simulink model "mano_buena_pinza_paper"  (R2025a)
settings: Solver=ode23  StartTime=0.0  StopTime=10.5  FixedStep=20e-3  MaxStep=1e-3  RelTol=1e-2  AbsTol=1e-4
model workspace: external: MATLAB File mano_vf_DataFile1.m (data not in the file)
undefined symbols (not defined in the file): smiData, X, Y, Z
libraries: sm_lib x268, nesl_utility x26
(part 3 of 7)

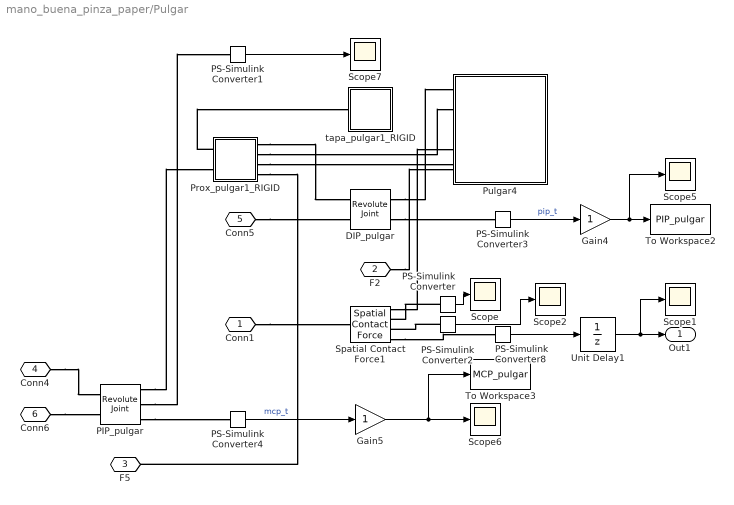
== system mano_buena_pinza_paper/Pulgar ==
  DIP_pulgar : sm_lib/Joints/Revolute Joint  JointMode=Normal  CompositeWrenchDir=FollowerOnBase  CompositeWrenchFrame=BaseFrame  SenseConstraintForce=off  SenseConstraintTorque=off  SenseTotalForce=off  SenseTotalTorque=off  PositionTargetSpecify=on  PositionTargetPriority=Low  PositionTargetValue=smiData.RevoluteJoint(41).Rz.Pos  PositionTargetValueUnits=deg  VelocityTargetSpecify=off  VelocityTargetPriority=High  VelocityTargetValue=0  VelocityTargetValueUnits=deg/s  EquilibriumPosition=0  EquilibriumPositionUnits=deg  SpringStiffness=0  SpringStiffnessUnits=N*m/deg  DampingCoefficient=0  DampingCoefficientUnits=N*m/(deg/s)  LowerLimitSpecify=off  LowerLimitBound=-90  LowerLimitBoundUnits=deg  LowerLimitStiffness=1e4  LowerLimitStiffnessUnits=N*m/deg  LowerLimitDamping=10  LowerLimitDampingUnits=N*m/(deg/s)  LowerLimitTransitionRegionWidth=0.1  LowerLimitTransitionRegionWidthUnits=deg  UpperLimitSpecify=off  UpperLimitBound=90  UpperLimitBoundUnits=deg  UpperLimitStiffness=1e4  UpperLimitStiffnessUnits=N*m/deg  UpperLimitDamping=10  UpperLimitDampingUnits=N*m/(deg/s)  UpperLimitTransitionRegionWidth=0.1  UpperLimitTransitionRegionWidthUnits=deg  TorqueActuationMode=ComputedTorque  MotionActuationMode=InputMotion  SensePosition=off  SenseVelocity=off  SenseAcceleration=off  SenseTorqueForce=on  SenseLowerLimitTorqueForce=off  SenseUpperLimitTorqueForce=off
  Gain4 : Gain
  Gain5 : Gain
  PIP_pulgar : sm_lib/Joints/Revolute Joint  JointMode=Normal  CompositeWrenchDir=FollowerOnBase  CompositeWrenchFrame=BaseFrame  SenseConstraintForce=off  SenseConstraintTorque=off  SenseTotalForce=off  SenseTotalTorque=off  PositionTargetSpecify=on  PositionTargetPriority=Low  PositionTargetValue=smiData.RevoluteJoint(36).Rz.Pos  PositionTargetValueUnits=deg  VelocityTargetSpecify=off  VelocityTargetPriority=High  VelocityTargetValue=0  VelocityTargetValueUnits=deg/s  EquilibriumPosition=0  EquilibriumPositionUnits=deg  SpringStiffness=0  SpringStiffnessUnits=N*m/deg  DampingCoefficient=0  DampingCoefficientUnits=N*m/(deg/s)  LowerLimitSpecify=off  LowerLimitBound=-90  LowerLimitBoundUnits=deg  LowerLimitStiffness=1e4  LowerLimitStiffnessUnits=N*m/deg  LowerLimitDamping=10  LowerLimitDampingUnits=N*m/(deg/s)  LowerLimitTransitionRegionWidth=0.1  LowerLimitTransitionRegionWidthUnits=deg  UpperLimitSpecify=off  UpperLimitBound=90  UpperLimitBoundUnits=deg  UpperLimitStiffness=1e4  UpperLimitStiffnessUnits=N*m/deg  UpperLimitDamping=10  UpperLimitDampingUnits=N*m/(deg/s)  UpperLimitTransitionRegionWidth=0.1  UpperLimitTransitionRegionWidthUnits=deg  TorqueActuationMode=ComputedTorque  MotionActuationMode=InputMotion  SensePosition=on  SenseVelocity=off  SenseAcceleration=off  SenseTorqueForce=on  SenseLowerLimitTorqueForce=off  SenseUpperLimitTorqueForce=off
  PS-Simulink Converter : nesl_utility/PS-Simulink Converter  PhysicalDomain=network_engine_domain  SubClassName=ps_output  LeftPortType=input  RightPortType=output  PseudoPeriodic=off  Frequencies=[]  VectorFormat=inherit  Unit=inherit  AffineConversion=off
  PS-Simulink Converter1 : nesl_utility/PS-Simulink Converter  PhysicalDomain=network_engine_domain  SubClassName=ps_output  LeftPortType=input  RightPortType=output  PseudoPeriodic=off  Frequencies=[]  VectorFormat=inherit  Unit=deg  AffineConversion=off
  PS-Simulink Converter2 : nesl_utility/PS-Simulink Converter  PhysicalDomain=network_engine_domain  SubClassName=ps_output  LeftPortType=input  RightPortType=output  PseudoPeriodic=off  Frequencies=[]  VectorFormat=inherit  Unit=mm  AffineConversion=off
  PS-Simulink Converter3 : nesl_utility/PS-Simulink Converter  PhysicalDomain=network_engine_domain  SubClassName=ps_output  LeftPortType=input  RightPortType=output  PseudoPeriodic=off  Frequencies=[]  VectorFormat=inherit  Unit=N*mm  AffineConversion=off
  PS-Simulink Converter4 : nesl_utility/PS-Simulink Converter  PhysicalDomain=network_engine_domain  SubClassName=ps_output  LeftPortType=input  RightPortType=output  PseudoPeriodic=off  Frequencies=[]  VectorFormat=inherit  Unit=N*mm  AffineConversion=off
  PS-Simulink Converter8 : nesl_utility/PS-Simulink Converter  PhysicalDomain=network_engine_domain  SubClassName=ps_output  LeftPortType=input  RightPortType=output  PseudoPeriodic=off  Frequencies=[]  VectorFormat=inherit  Unit=N  AffineConversion=off
  Prox_pulgar1_RIGID : Subsystem
  Pulgar4 : Subsystem
  Scope{,1..2,5..7} (6 alike) : Scope
      Scope settings: DataLoggingVariableName=ScopeData15
      Scope1 settings: ActiveDisplayYMinimum=-0.19095791938029771  ActiveDisplayYMaximum=2.3213655450923372
      Scope2 settings: DataLoggingVariableName=ScopeData16
      Scope5 settings: ActiveDisplayYMinimum=-74.001415056347014  ActiveDisplayYMaximum=341.55104024365312  DataLoggingVariableName=ScopeData5
      Scope6 settings: ActiveDisplayYMinimum=-154.71464722510333  ActiveDisplayYMaximum=184.74085697959597  DataLoggingVariableName=ScopeData6
      Scope7 settings: ActiveDisplayYMinimum=-1  ActiveDisplayYMaximum=1  DataLoggingVariableName=ScopeData7
  Spatial Contact Force1 : sm_lib/Forces and Torques/Spatial Contact Force  SenseSeparationDistance=off  NormalForceType=SmoothSpringDamper  NormalStiffness=2e4  NormalStiffnessUnits=N/m  NormalDamping=30  NormalDampingUnits=N/(m/s)  NormalTransitionRegionWidth=1e-3  NormalTransitionRegionWidthUnits=m  FrictionType=SmoothStickSlip  CoefficientOfStaticFriction=0.5  CoefficientOfDynamicFriction=0.3  FrictionalCriticalVelocity=1e-2  FrictionalCriticalVelocityUnits=m/s  SenseContactSignal=on  SensePenetrationDepth=on  SenseNormalVelocity=off  SenseTangentialVelocity=off  SensingForceTorqueDirection=BaseOnFollower  SensingForceTorqueResolutionFrame=ContactFrame  SenseNormalForce=off  SenseNormalForceMagnitude=on  SenseNormalTorque=off  SenseFrictionalForce=off  SenseFrictionalForceMagnitude=off  SenseFrictionalTorque=off  SenseTotalForce=off  SenseTotalTorque=off  SenseContactBaseRotation=off  SenseContactBaseTranslation=off  SenseContactFollowerRotation=off  SenseContactFollowerTranslation=off  ZeroCrossDetectContactStartAndEnd=off
  To Workspace2 : ToWorkspace  VariableName=PIP_pulgar  SaveFormat=Timeseries  SampleTime=-1
  To Workspace3 : ToWorkspace  VariableName=MCP_pulgar  SaveFormat=Timeseries  SampleTime=-1
  Unit Delay1 : UnitDelay  SampleTime=20e-3  HasFrameUpgradeWarning=on
  tapa_pulgar1_RIGID : Subsystem
  Conn1 : PMIOPort  Side=Left
  F2 : PMIOPort  Port=2  Side=Left
  F5 : PMIOPort  Port=3  Side=Right
  Conn4 : PMIOPort  Port=4  Side=Left
  Conn5 : PMIOPort  Port=5  Side=Left
  Conn6 : PMIOPort  Port=6  Side=Left
  Out1 : Outport
  wires:
  PS-Simulink Converter1/1 -> Scope7/1
  PS-Simulink Converter4/1 -> Gain5/1  "mcp_t"
  Gain5/1 -> To Workspace3/1, Scope6/1
  PS-Simulink Converter3/1 -> Gain4/1  "pip_t"
  PS-Simulink Converter8/1 -> Unit Delay1/1
  Gain4/1 -> To Workspace2/1, Scope5/1
  Unit Delay1/1 -> Scope1/1, Out1/1
  PS-Simulink Converter/1 -> Scope/1
  PS-Simulink Converter2/1 -> Scope2/1
  connections:
  Conn6/RConn1 -- PIP_pulgar/LConn2
  Conn4/RConn1 -- PIP_pulgar/LConn1
  DIP_pulgar/RConn1 -- Pulgar4/LConn1
  Prox_pulgar1_RIGID/LConn1 -- tapa_pulgar1_RIGID/LConn1
  PIP_pulgar/RConn1 -- Prox_pulgar1_RIGID/LConn2
  PIP_pulgar/RConn2 -- PS-Simulink Converter1/LConn1
  Prox_pulgar1_RIGID/RConn1 -- DIP_pulgar/LConn1
  PIP_pulgar/RConn3 -- PS-Simulink Converter4/LConn1
  Prox_pulgar1_RIGID/RConn4 -- F5/RConn1
  Prox_pulgar1_RIGID/RConn2 -- Pulgar4/LConn2
  Prox_pulgar1_RIGID/RConn3 -- Pulgar4/LConn3
  Conn5/RConn1 -- DIP_pulgar/LConn2
  Conn1/RConn1 -- Spatial Contact Force1/LConn1
  DIP_pulgar/RConn2 -- PS-Simulink Converter3/LConn1
  F2/RConn1 -- Pulgar4/LConn5
  Spatial Contact Force1/RConn1 -- Pulgar4/LConn4
  Spatial Contact Force1/RConn4 -- PS-Simulink Converter8/LConn1
  PS-Simulink Converter/LConn1 -- Spatial Contact Force1/RConn2
  PS-Simulink Converter2/LConn1 -- Spatial Contact Force1/RConn3

== system mano_buena_pinza_paper/Subsystem ==
  Angulo_ref : Inport
  Demux1 : Demux  Outputs=2
  Discrete State-Space : DiscreteStateSpace  A=[1 0.0196;0 0.9604]  B=[1e-4*0.0051;1e-4*0.5045]  C=eye(2)  D=[0 ;0]  SampleTime=20e-3
  Gain : Gain  Gain=pi/180
  Gain1 : Gain  Gain=1000
  Gain4 : Gain  Gain=180/pi
  Gain5 : Gain  Gain=[2192.4 757.4]  Multiplication=Matrix(K*u) (u vector)
  Saturation : Saturate  UpperLimit=4095  LowerLimit=-4095
  Scope1 : Scope
      settings: ActiveDisplayYMinimum=-514.3876517918344  ActiveDisplayYMaximum=3883.614035604794  DataLoggingVariableName=ScopeData8
  Scope6 : Scope
      settings: ActiveDisplayYMinimum=-70.37229560740974  ActiveDisplayYMaximum=586.35935668183049  DataLoggingVariableName=ScopeData11
  Sum : Sum  Inputs=|+-
  Angulo_real : Outport
  wires:
  Gain5/1 -> Saturation/1
  Discrete State-Space/1 -> Demux1/1, Sum/2  "LQR"
  Sum/1 -> Gain5/1
  Saturation/1 -> Scope1/1, Discrete State-Space/1
  Demux1/1 -> Gain4/1
  Angulo_ref/1 -> Gain/1
  Demux1/2 -> Gain1/1
  Gain4/1 -> Angulo_real/1
  Gain/1 -> Sum/1
  Gain1/1 -> Scope6/1

== system mano_buena_pinza_paper/Subsystem1 ==
  Angulo_ref : Inport
  Demux1 : Demux  Outputs=2
  Discrete State-Space : DiscreteStateSpace  A=[1 0.0196;0 0.9604]  B=[1e-4*0.0051;1e-4*0.5045]  C=eye(2)  D=[0 ;0]  SampleTime=20e-3
  Gain : Gain  Gain=pi/180
  Gain1 : Gain  Gain=1000
  Gain4 : Gain  Gain=180/pi
  Gain5 : Gain  Gain=[2192.4 757.4]  Multiplication=Matrix(K*u) (u vector)
  Saturation : Saturate  UpperLimit=4095  LowerLimit=-4095
  Scope1 : Scope
      settings: ActiveDisplayYMinimum=-514.3876517918344  ActiveDisplayYMaximum=3883.614035604794  DataLoggingVariableName=ScopeData8
  Scope6 : Scope
      settings: ActiveDisplayYMinimum=-178.26281177195131  ActiveDisplayYMaximum=1149.4351414549326  DataLoggingVariableName=ScopeData11
  Sum : Sum  Inputs=|+-
  Angulo_real : Outport
  wires:
  Gain5/1 -> Saturation/1
  Discrete State-Space/1 -> Demux1/1, Sum/2  "LQR"
  Sum/1 -> Gain5/1
  Saturation/1 -> Scope1/1, Discrete State-Space/1
  Demux1/1 -> Gain4/1
  Angulo_ref/1 -> Gain/1
  Demux1/2 -> Gain1/1
  Gain4/1 -> Angulo_real/1
  Gain/1 -> Sum/1
  Gain1/1 -> Scope6/1

== system mano_buena_pinza_paper/Subsystem2 ==
  Angulo_ref : Inport
  Demux1 : Demux  Outputs=2
  Discrete State-Space : DiscreteStateSpace  A=[1 0.0196;0 0.9604]  B=[1e-4*0.0051;1e-4*0.5045]  C=eye(2)  D=[0 ;0]  SampleTime=20e-3
  Gain : Gain  Gain=pi/180
  Gain4 : Gain  Gain=180/pi
  Gain5 : Gain  Gain=[2192.4 757.4]  Multiplication=Matrix(K*u) (u vector)
  Saturation : Saturate  UpperLimit=4095  LowerLimit=-4095
  Scope1 : Scope
      settings: ActiveDisplayYMinimum=-514.3876517918344  ActiveDisplayYMaximum=3883.614035604794  DataLoggingVariableName=ScopeData8
  Scope6 : Scope
      settings: ActiveDisplayYMinimum=-0.21091417850221092  ActiveDisplayYMaximum=1.7573278410890731  DataLoggingVariableName=ScopeData11
  Sum : Sum  Inputs=|+-
  Angulo_real : Outport
  wires:
  Gain5/1 -> Saturation/1
  Discrete State-Space/1 -> Demux1/1, Sum/2  "LQR"
  Sum/1 -> Gain5/1
  Saturation/1 -> Scope1/1, Discrete State-Space/1
  Demux1/1 -> Gain4/1
  Angulo_ref/1 -> Gain/1
  Demux1/2 -> Scope6/1
  Gain4/1 -> Angulo_real/1
  Gain/1 -> Sum/1

== system mano_buena_pinza_paper/Subsystem3 ==
  Angulo_ref : Inport
  Demux1 : Demux  Outputs=2
  Discrete State-Space : DiscreteStateSpace  A=[1 0.0196;0 0.9604]  B=[1e-4*0.0051;1e-4*0.5045]  C=eye(2)  D=[0 ;0]  SampleTime=20e-3
  Gain : Gain  Gain=pi/180
  Gain4 : Gain  Gain=180/pi
  Gain5 : Gain  Gain=[2192.4 757.4]  Multiplication=Matrix(K*u) (u vector)
  Saturation : Saturate  UpperLimit=4095  LowerLimit=-4095
  Scope1 : Scope
      settings: ActiveDisplayYMinimum=-514.3876517918344  ActiveDisplayYMaximum=3883.614035604794  DataLoggingVariableName=ScopeData8
  Scope6 : Scope
      settings: ActiveDisplayYMinimum=-0.21091417850221092  ActiveDisplayYMaximum=1.7573278410890731  DataLoggingVariableName=ScopeData11
  Sum : Sum  Inputs=|+-
  Angulo_real : Outport
  wires:
  Gain5/1 -> Saturation/1
  Discrete State-Space/1 -> Demux1/1, Sum/2  "LQR"
  Sum/1 -> Gain5/1
  Saturation/1 -> Scope1/1, Discrete State-Space/1
  Demux1/1 -> Gain4/1
  Angulo_ref/1 -> Gain/1
  Demux1/2 -> Scope6/1
  Gain4/1 -> Angulo_real/1
  Gain/1 -> Sum/1

== system mano_buena_pinza_paper/Subsystem4 ==
  Angulo_ref : Inport
  Demux1 : Demux  Outputs=2
  Discrete State-Space : DiscreteStateSpace  A=[1 0.0196;0 0.9604]  B=[1e-4*0.0051;1e-4*0.5045]  C=eye(2)  D=[0 ;0]  SampleTime=20e-3
  Gain : Gain  Gain=pi/180
  Gain4 : Gain  Gain=180/pi
  Gain5 : Gain  Gain=[2192.4 757.4]  Multiplication=Matrix(K*u) (u vector)
  Saturation : Saturate  UpperLimit=4095  LowerLimit=-4095
  Scope1 : Scope
      settings: ActiveDisplayYMinimum=-514.3876517918344  ActiveDisplayYMaximum=3883.614035604794  DataLoggingVariableName=ScopeData8
  Scope6 : Scope
      settings: ActiveDisplayYMinimum=-0.21091417850221092  ActiveDisplayYMaximum=1.7573278410890731  DataLoggingVariableName=ScopeData11
  Sum : Sum  Inputs=|+-
  Angulo_real : Outport
  wires:
  Gain5/1 -> Saturation/1
  Discrete State-Space/1 -> Demux1/1, Sum/2  "LQR"
  Sum/1 -> Gain5/1
  Saturation/1 -> Scope1/1, Discrete State-Space/1
  Demux1/1 -> Gain4/1
  Angulo_ref/1 -> Gain/1
  Demux1/2 -> Scope6/1
  Gain4/1 -> Angulo_real/1
  Gain/1 -> Sum/1

== system mano_buena_pinza_paper/Subsystem5 ==
  Angulo_ref : Inport
  Demux1 : Demux  Outputs=2
  Discrete State-Space : DiscreteStateSpace  A=[1 0.0196;0 0.9604]  B=[1e-4*0.0051;1e-4*0.5045]  C=eye(2)  D=[0 ;0]  SampleTime=20e-3
  Gain : Gain  Gain=pi/180
  Gain4 : Gain  Gain=180/pi
  Gain5 : Gain  Gain=[2192.4 757.4]  Multiplication=Matrix(K*u) (u vector)
  Saturation : Saturate  UpperLimit=4095  LowerLimit=-4095
  Scope1 : Scope
      settings: ActiveDisplayYMinimum=-514.3876517918344  ActiveDisplayYMaximum=3883.614035604794  DataLoggingVariableName=ScopeData8
  Scope6 : Scope
      settings: ActiveDisplayYMinimum=-0.21091417850221092  ActiveDisplayYMaximum=1.7573278410890731  DataLoggingVariableName=ScopeData11
  Sum : Sum  Inputs=|+-
  Angulo_real : Outport
  wires:
  Gain5/1 -> Saturation/1
  Discrete State-Space/1 -> Demux1/1, Sum/2  "LQR"
  Sum/1 -> Gain5/1
  Saturation/1 -> Scope1/1, Discrete State-Space/1
  Demux1/1 -> Gain4/1
  Angulo_ref/1 -> Gain/1
  Demux1/2 -> Scope6/1
  Gain4/1 -> Angulo_real/1
  Gain/1 -> Sum/1

== system mano_buena_pinza_paper/Subsystem6 ==
  Angulo_ref : Inport
  Demux1 : Demux  Outputs=2
  Discrete State-Space : DiscreteStateSpace  A=[1 0.0196;0 0.9604]  B=[1e-4*0.0051;1e-4*0.5045]  C=eye(2)  D=[0 ;0]  SampleTime=20e-3
  Gain : Gain  Gain=pi/180
  Gain4 : Gain  Gain=180/pi
  Gain5 : Gain  Gain=[2192.4 757.4]  Multiplication=Matrix(K*u) (u vector)
  Saturation : Saturate  UpperLimit=4095  LowerLimit=-4095
  Scope1 : Scope
      settings: ActiveDisplayYMinimum=-514.3876517918344  ActiveDisplayYMaximum=3883.614035604794  DataLoggingVariableName=ScopeData8
  Scope6 : Scope
      settings: ActiveDisplayYMinimum=-0.21091417850221092  ActiveDisplayYMaximum=1.7573278410890731  DataLoggingVariableName=ScopeData11
  Sum : Sum  Inputs=|+-
  Angulo_real : Outport
  wires:
  Gain5/1 -> Saturation/1
  Discrete State-Space/1 -> Demux1/1, Sum/2  "LQR"
  Sum/1 -> Gain5/1
  Saturation/1 -> Scope1/1, Discrete State-Space/1
  Demux1/1 -> Gain4/1
  Angulo_ref/1 -> Gain/1
  Demux1/2 -> Scope6/1
  Gain4/1 -> Angulo_real/1
  Gain/1 -> Sum/1

== system mano_buena_pinza_paper/Subsystem7 ==
  Angulo_ref : Inport
  Demux1 : Demux  Outputs=2
  Discrete State-Space : DiscreteStateSpace  A=[1 0.0196;0 0.9604]  B=[1e-4*0.0051;1e-4*0.5045]  C=eye(2)  D=[0 ;0]  SampleTime=20e-3
  Gain : Gain  Gain=pi/180
  Gain4 : Gain  Gain=180/pi
  Gain5 : Gain  Gain=[2192.4 757.4]  Multiplication=Matrix(K*u) (u vector)
  Saturation : Saturate  UpperLimit=4095  LowerLimit=-4095
  Scope1 : Scope
      settings: ActiveDisplayYMinimum=-514.3876517918344  ActiveDisplayYMaximum=3883.614035604794  DataLoggingVariableName=ScopeData8
  Scope6 : Scope
      settings: ActiveDisplayYMinimum=-0.21091417850221092  ActiveDisplayYMaximum=1.7573278410890731  DataLoggingVariableName=ScopeData11
  Sum : Sum  Inputs=|+-
  Angulo_real : Outport
  wires:
  Gain5/1 -> Saturation/1
  Discrete State-Space/1 -> Demux1/1, Sum/2  "LQR"
  Sum/1 -> Gain5/1
  Saturation/1 -> Scope1/1, Discrete State-Space/1
  Demux1/1 -> Gain4/1
  Angulo_ref/1 -> Gain/1
  Demux1/2 -> Scope6/1
  Gain4/1 -> Angulo_real/1
  Gain/1 -> Sum/1

== system mano_buena_pinza_paper/Subsystem8 ==
  Angulo_ref : Inport
  Demux1 : Demux  Outputs=2
  Discrete State-Space : DiscreteStateSpace  A=[1 0.0196;0 0.9604]  B=[1e-4*0.0051;1e-4*0.5045]  C=eye(2)  D=[0 ;0]  SampleTime=20e-3
  Gain : Gain  Gain=pi/180
  Gain4 : Gain  Gain=180/pi
  Gain5 : Gain  Gain=[2192.4 757.4]  Multiplication=Matrix(K*u) (u vector)
  Saturation : Saturate  UpperLimit=4095  LowerLimit=-4095
  Scope1 : Scope
      settings: ActiveDisplayYMinimum=-514.3876517918344  ActiveDisplayYMaximum=3883.614035604794  DataLoggingVariableName=ScopeData8
  Scope6 : Scope
      settings: ActiveDisplayYMinimum=-0.21091417850221092  ActiveDisplayYMaximum=1.7573278410890731  DataLoggingVariableName=ScopeData11
  Sum : Sum  Inputs=|+-
  Angulo_real : Outport
  wires:
  Gain5/1 -> Saturation/1
  Discrete State-Space/1 -> Demux1/1, Sum/2  "LQR"
  Sum/1 -> Gain5/1
  Saturation/1 -> Scope1/1, Discrete State-Space/1
  Demux1/1 -> Gain4/1
  Angulo_ref/1 -> Gain/1
  Demux1/2 -> Scope6/1
  Gain4/1 -> Angulo_real/1
  Gain/1 -> Sum/1

== system mano_buena_pinza_paper/Subsystem9 ==
  Angulo_ref : Inport
  Demux1 : Demux  Outputs=2
  Discrete State-Space : DiscreteStateSpace  A=[1 0.0196;0 0.9604]  B=[1e-4*0.0051;1e-4*0.5045]  C=eye(2)  D=[0 ;0]  SampleTime=20e-3
  Gain : Gain  Gain=pi/180
  Gain4 : Gain  Gain=180/pi
  Gain5 : Gain  Gain=[2192.4 757.4]  Multiplication=Matrix(K*u) (u vector)
  Saturation : Saturate  UpperLimit=4095  LowerLimit=-4095
  Scope1 : Scope
      settings: ActiveDisplayYMinimum=-514.3876517918344  ActiveDisplayYMaximum=3883.614035604794  DataLoggingVariableName=ScopeData8
  Scope6 : Scope
      settings: ActiveDisplayYMinimum=-0.21091417850221092  ActiveDisplayYMaximum=1.7573278410890731  DataLoggingVariableName=ScopeData11
  Sum : Sum  Inputs=|+-
  Angulo_real : Outport
  wires:
  Gain5/1 -> Saturation/1
  Discrete State-Space/1 -> Demux1/1, Sum/2  "LQR"
  Sum/1 -> Gain5/1
  Saturation/1 -> Scope1/1, Discrete State-Space/1
  Demux1/1 -> Gain4/1
  Angulo_ref/1 -> Gain/1
  Demux1/2 -> Scope6/1
  Gain4/1 -> Angulo_real/1
  Gain/1 -> Sum/1

== system mano_buena_pinza_paper/Tapa_meta_indice2_RIGID ==
  ReferenceFrame : sm_lib/Frames and Transforms/Reference Frame
  Solid : sm_lib/Body Elements/File Solid  ExtGeomFileName=Tapa_meta_indice_ipt_ad682b4a.STEP  UnitType=FromFile  ExtGeomFileUnits=m  StepReaderType=HEX  ExportConvexHullGeometry=off  InertiaType=Custom  BasedOnType=DensityFromFile  Density=1000  DensityUnits=kg/m^3  Mass=smiData.Solid(12).mass  MassUnits=kg  CenterOfMass=smiData.Solid(12).CoM  CenterOfMassUnits=mm  MomentsOfInertia=smiData.Solid(12).MoI  MomentsOfInertiaUnits=kg*mm^2  ProductsOfInertia=smiData.Solid(12).PoI  ProductsOfInertiaUnits=kg*mm^2  GraphicType=FromGeometry  MarkerShape=Sphere  MarkerSize=10  GraphicVisPropType=SimpleVisualProperties  GraphicDiffuseColor=smiData.Solid(12).color  GraphicOpacity=smiData.Solid(12).opacity  GraphicSpecularColor=[0.5 0.5 0.5 1.0]  GraphicAmbientColor=[0.15 0.15 0.15 1.0]  GraphicEmissiveColor=[0.0 0.0 0.0 1.0]  GraphicShininess=75  DoExposeReferenceFrame=on  SerializedFrames=<Frames/>
  Transform : sm_lib/Frames and Transforms/Rigid Transform  RotationMethod=ArbitraryAxis  FollAlignAxisA=+X  BaseAlignAxisA=+Y  FollAlignAxisB=+Y  BaseAlignAxisB=+Z  RotationStandardAxis=+Z  RotationAngle=smiData.RigidTransform(94).angle  RotationAngleUnits=rad  RotationArbitraryAxis=smiData.RigidTransform(94).axis  RotationSequenceAxes=FollowerAxes  RotationSequence=XYX  RotationSequenceAngles=[0 0 0]  RotationSequenceAnglesUnits=deg  RotationMatrix=[1 0 0;0 1 0;0 0 1]  Quaternion=[1 0 0 0]  TranslationMethod=Cartesian  TranslationCartesianOffset=smiData.RigidTransform(94).translation  TranslationCartesianOffsetUnits=mm  TranslationStandardAxis=+Z  TranslationStandardOffset=0  TranslationStandardOffsetUnits=m  TranslationROffset=0  TranslationROffsetUnits=m  TranslationThetaOffset=0  TranslationThetaOffsetUnits=deg  TranslationZOffset=0  TranslationZOffsetUnits=m
  F : PMIOPort  Side=Left
  connections:
  Solid/RConn1 -- ReferenceFrame/RConn1 -- Transform/LConn1
  Transform/RConn1 -- F/RConn1

== system mano_buena_pinza_paper/Tapa_meta_indice3_RIGID ==
  ReferenceFrame : sm_lib/Frames and Transforms/Reference Frame
  Solid : sm_lib/Body Elements/File Solid  ExtGeomFileName=Tapa_meta_indice_ipt_ad682b4a.STEP  UnitType=FromFile  ExtGeomFileUnits=m  StepReaderType=HEX  ExportConvexHullGeometry=off  InertiaType=Custom  BasedOnType=DensityFromFile  Density=1000  DensityUnits=kg/m^3  Mass=smiData.Solid(12).mass  MassUnits=kg  CenterOfMass=smiData.Solid(12).CoM  CenterOfMassUnits=mm  MomentsOfInertia=smiData.Solid(12).MoI  MomentsOfInertiaUnits=kg*mm^2  ProductsOfInertia=smiData.Solid(12).PoI  ProductsOfInertiaUnits=kg*mm^2  GraphicType=FromGeometry  MarkerShape=Sphere  MarkerSize=10  GraphicVisPropType=SimpleVisualProperties  GraphicDiffuseColor=smiData.Solid(12).color  GraphicOpacity=smiData.Solid(12).opacity  GraphicSpecularColor=[0.5 0.5 0.5 1.0]  GraphicAmbientColor=[0.15 0.15 0.15 1.0]  GraphicEmissiveColor=[0.0 0.0 0.0 1.0]  GraphicShininess=75  DoExposeReferenceFrame=on  SerializedFrames=<Frames/>
  Transform : sm_lib/Frames and Transforms/Rigid Transform  RotationMethod=ArbitraryAxis  FollAlignAxisA=+X  BaseAlignAxisA=+Y  FollAlignAxisB=+Y  BaseAlignAxisB=+Z  RotationStandardAxis=+Z  RotationAngle=smiData.RigidTransform(95).angle  RotationAngleUnits=rad  RotationArbitraryAxis=smiData.RigidTransform(95).axis  RotationSequenceAxes=FollowerAxes  RotationSequence=XYX  RotationSequenceAngles=[0 0 0]  RotationSequenceAnglesUnits=deg  RotationMatrix=[1 0 0;0 1 0;0 0 1]  Quaternion=[1 0 0 0]  TranslationMethod=Cartesian  TranslationCartesianOffset=smiData.RigidTransform(95).translation  TranslationCartesianOffsetUnits=mm  TranslationStandardAxis=+Z  TranslationStandardOffset=0  TranslationStandardOffsetUnits=m  TranslationROffset=0  TranslationROffsetUnits=m  TranslationThetaOffset=0  TranslationThetaOffsetUnits=deg  TranslationZOffset=0  TranslationZOffsetUnits=m
  Transform1 : sm_lib/Frames and Transforms/Rigid Transform  RotationMethod=ArbitraryAxis  FollAlignAxisA=+X  BaseAlignAxisA=+Y  FollAlignAxisB=+Y  BaseAlignAxisB=+Z  RotationStandardAxis=+Z  RotationAngle=smiData.RigidTransform(107).angle  RotationAngleUnits=rad  RotationArbitraryAxis=smiData.RigidTransform(107).axis  RotationSequenceAxes=FollowerAxes  RotationSequence=XYX  RotationSequenceAngles=[0 0 0]  RotationSequenceAnglesUnits=deg  RotationMatrix=[1 0 0;0 1 0;0 0 1]  Quaternion=[1 0 0 0]  TranslationMethod=Cartesian  TranslationCartesianOffset=smiData.RigidTransform(107).translation  TranslationCartesianOffsetUnits=mm  TranslationStandardAxis=+Z  TranslationStandardOffset=0  TranslationStandardOffsetUnits=m  TranslationROffset=0  TranslationROffsetUnits=m  TranslationThetaOffset=0  TranslationThetaOffsetUnits=deg  TranslationZOffset=0  TranslationZOffsetUnits=m
  F : PMIOPort  Side=Left
  F1 : PMIOPort  Port=2  Side=Right
  connections:
  Solid/RConn1 -- ReferenceFrame/RConn1 -- Transform/LConn1 -- Transform1/LConn1
  Transform/RConn1 -- F/RConn1
  Transform1/RConn1 -- F1/RConn1

== system mano_buena_pinza_paper/Tapa_meta_indice4_RIGID ==
  ReferenceFrame : sm_lib/Frames and Transforms/Reference Frame
  Solid : sm_lib/Body Elements/File Solid  ExtGeomFileName=Tapa_meta_indice_ipt_ad682b4a.STEP  UnitType=FromFile  ExtGeomFileUnits=m  StepReaderType=HEX  ExportConvexHullGeometry=off  InertiaType=Custom  BasedOnType=DensityFromFile  Density=1000  DensityUnits=kg/m^3  Mass=smiData.Solid(12).mass  MassUnits=kg  CenterOfMass=smiData.Solid(12).CoM  CenterOfMassUnits=mm  MomentsOfInertia=smiData.Solid(12).MoI  MomentsOfInertiaUnits=kg*mm^2  ProductsOfInertia=smiData.Solid(12).PoI  ProductsOfInertiaUnits=kg*mm^2  GraphicType=FromGeometry  MarkerShape=Sphere  MarkerSize=10  GraphicVisPropType=SimpleVisualProperties  GraphicDiffuseColor=smiData.Solid(12).color  GraphicOpacity=smiData.Solid(12).opacity  GraphicSpecularColor=[0.5 0.5 0.5 1.0]  GraphicAmbientColor=[0.15 0.15 0.15 1.0]  GraphicEmissiveColor=[0.0 0.0 0.0 1.0]  GraphicShininess=75  DoExposeReferenceFrame=on  SerializedFrames=<Frames/>
  Transform : sm_lib/Frames and Transforms/Rigid Transform  RotationMethod=ArbitraryAxis  FollAlignAxisA=+X  BaseAlignAxisA=+Y  FollAlignAxisB=+Y  BaseAlignAxisB=+Z  RotationStandardAxis=+Z  RotationAngle=smiData.RigidTransform(97).angle  RotationAngleUnits=rad  RotationArbitraryAxis=smiData.RigidTransform(97).axis  RotationSequenceAxes=FollowerAxes  RotationSequence=XYX  RotationSequenceAngles=[0 0 0]  RotationSequenceAnglesUnits=deg  RotationMatrix=[1 0 0;0 1 0;0 0 1]  Quaternion=[1 0 0 0]  TranslationMethod=Cartesian  TranslationCartesianOffset=smiData.RigidTransform(97).translation  TranslationCartesianOffsetUnits=mm  TranslationStandardAxis=+Z  TranslationStandardOffset=0  TranslationStandardOffsetUnits=m  TranslationROffset=0  TranslationROffsetUnits=m  TranslationThetaOffset=0  TranslationThetaOffsetUnits=deg  TranslationZOffset=0  TranslationZOffsetUnits=m
  F : PMIOPort  Side=Left
  connections:
  Solid/RConn1 -- ReferenceFrame/RConn1 -- Transform/LConn1
  Transform/RConn1 -- F/RConn1

== system mano_buena_pinza_paper/Abduccion_4/Esl21_RIGID ==
  ReferenceFrame : sm_lib/Frames and Transforms/Reference Frame
  Solid : sm_lib/Body Elements/File Solid  ExtGeomFileName=Esl2_ipt_5f6dfdfa.STEP  UnitType=FromFile  ExtGeomFileUnits=m  StepReaderType=HEX  ExportConvexHullGeometry=off  InertiaType=Custom  BasedOnType=DensityFromFile  Density=1000  DensityUnits=kg/m^3  Mass=smiData.Solid(31).mass  MassUnits=kg  CenterOfMass=smiData.Solid(31).CoM  CenterOfMassUnits=mm  MomentsOfInertia=smiData.Solid(31).MoI  MomentsOfInertiaUnits=kg*mm^2  ProductsOfInertia=smiData.Solid(31).PoI  ProductsOfInertiaUnits=kg*mm^2  GraphicType=FromGeometry  MarkerShape=Sphere  MarkerSize=10  GraphicVisPropType=SimpleVisualProperties  GraphicDiffuseColor=smiData.Solid(31).color  GraphicOpacity=smiData.Solid(31).opacity  GraphicSpecularColor=[0.5 0.5 0.5 1.0]  GraphicAmbientColor=[0.15 0.15 0.15 1.0]  GraphicEmissiveColor=[0.0 0.0 0.0 1.0]  GraphicShininess=75  DoExposeReferenceFrame=on  SerializedFrames=<Frames/>
  Transform : sm_lib/Frames and Transforms/Rigid Transform  RotationMethod=ArbitraryAxis  FollAlignAxisA=+X  BaseAlignAxisA=+Y  FollAlignAxisB=+Y  BaseAlignAxisB=+Z  RotationStandardAxis=+Z  RotationAngle=smiData.RigidTransform(42).angle  RotationAngleUnits=rad  RotationArbitraryAxis=smiData.RigidTransform(42).axis  RotationSequenceAxes=FollowerAxes  RotationSequence=XYX  RotationSequenceAngles=[0 0 0]  RotationSequenceAnglesUnits=deg  RotationMatrix=[1 0 0;0 1 0;0 0 1]  Quaternion=[1 0 0 0]  TranslationMethod=Cartesian  TranslationCartesianOffset=smiData.RigidTransform(42).translation  TranslationCartesianOffsetUnits=mm  TranslationStandardAxis=+Z  TranslationStandardOffset=0  TranslationStandardOffsetUnits=m  TranslationROffset=0  TranslationROffsetUnits=m  TranslationThetaOffset=0  TranslationThetaOffsetUnits=deg  TranslationZOffset=0  TranslationZOffsetUnits=m
  Transform1 : sm_lib/Frames and Transforms/Rigid Transform  RotationMethod=ArbitraryAxis  FollAlignAxisA=+X  BaseAlignAxisA=+Y  FollAlignAxisB=+Y  BaseAlignAxisB=+Z  RotationStandardAxis=+Z  RotationAngle=smiData.RigidTransform(44).angle  RotationAngleUnits=rad  RotationArbitraryAxis=smiData.RigidTransform(44).axis  RotationSequenceAxes=FollowerAxes  RotationSequence=XYX  RotationSequenceAngles=[0 0 0]  RotationSequenceAnglesUnits=deg  RotationMatrix=[1 0 0;0 1 0;0 0 1]  Quaternion=[1 0 0 0]  TranslationMethod=Cartesian  TranslationCartesianOffset=smiData.RigidTransform(44).translation  TranslationCartesianOffsetUnits=mm  TranslationStandardAxis=+Z  TranslationStandardOffset=0  TranslationStandardOffsetUnits=m  TranslationROffset=0  TranslationROffsetUnits=m  TranslationThetaOffset=0  TranslationThetaOffsetUnits=deg  TranslationZOffset=0  TranslationZOffsetUnits=m
  F1 : PMIOPort  Side=Left
  F : PMIOPort  Port=2  Side=Left
  connections:
  Solid/RConn1 -- ReferenceFrame/RConn1 -- Transform/LConn1 -- Transform1/LConn1
  Transform/RConn1 -- F/RConn1
  Transform1/RConn1 -- F1/RConn1

== system mano_buena_pinza_paper/Abduccion_4/Esl31_RIGID ==
  ReferenceFrame : sm_lib/Frames and Transforms/Reference Frame
  Solid : sm_lib/Body Elements/File Solid  ExtGeomFileName=Esl3_ipt_c845c934.STEP  UnitType=FromFile  ExtGeomFileUnits=m  StepReaderType=HEX  ExportConvexHullGeometry=off  InertiaType=Custom  BasedOnType=DensityFromFile  Density=1000  DensityUnits=kg/m^3  Mass=smiData.Solid(32).mass  MassUnits=kg  CenterOfMass=smiData.Solid(32).CoM  CenterOfMassUnits=mm  MomentsOfInertia=smiData.Solid(32).MoI  MomentsOfInertiaUnits=kg*mm^2  ProductsOfInertia=smiData.Solid(32).PoI  ProductsOfInertiaUnits=kg*mm^2  GraphicType=FromGeometry  MarkerShape=Sphere  MarkerSize=10  GraphicVisPropType=SimpleVisualProperties  GraphicDiffuseColor=smiData.Solid(32).color  GraphicOpacity=smiData.Solid(32).opacity  GraphicSpecularColor=[0.5 0.5 0.5 1.0]  GraphicAmbientColor=[0.15 0.15 0.15 1.0]  GraphicEmissiveColor=[0.0 0.0 0.0 1.0]  GraphicShininess=75  DoExposeReferenceFrame=on  SerializedFrames=<Frames/>
  Transform : sm_lib/Frames and Transforms/Rigid Transform  RotationMethod=ArbitraryAxis  FollAlignAxisA=+X  BaseAlignAxisA=+Y  FollAlignAxisB=+Y  BaseAlignAxisB=+Z  RotationStandardAxis=+Z  RotationAngle=smiData.RigidTransform(41).angle  RotationAngleUnits=rad  RotationArbitraryAxis=smiData.RigidTransform(41).axis  RotationSequenceAxes=FollowerAxes  RotationSequence=XYX  RotationSequenceAngles=[0 0 0]  RotationSequenceAnglesUnits=deg  RotationMatrix=[1 0 0;0 1 0;0 0 1]  Quaternion=[1 0 0 0]  TranslationMethod=Cartesian  TranslationCartesianOffset=smiData.RigidTransform(41).translation  TranslationCartesianOffsetUnits=mm  TranslationStandardAxis=+Z  TranslationStandardOffset=0  TranslationStandardOffsetUnits=m  TranslationROffset=0  TranslationROffsetUnits=m  TranslationThetaOffset=0  TranslationThetaOffsetUnits=deg  TranslationZOffset=0  TranslationZOffsetUnits=m
  Transform1 : sm_lib/Frames and Transforms/Rigid Transform  RotationMethod=ArbitraryAxis  FollAlignAxisA=+X  BaseAlignAxisA=+Y  FollAlignAxisB=+Y  BaseAlignAxisB=+Z  RotationStandardAxis=+Z  RotationAngle=smiData.RigidTransform(45).angle  RotationAngleUnits=rad  RotationArbitraryAxis=smiData.RigidTransform(45).axis  RotationSequenceAxes=FollowerAxes  RotationSequence=XYX  RotationSequenceAngles=[0 0 0]  RotationSequenceAnglesUnits=deg  RotationMatrix=[1 0 0;0 1 0;0 0 1]  Quaternion=[1 0 0 0]  TranslationMethod=Cartesian  TranslationCartesianOffset=smiData.RigidTransform(45).translation  TranslationCartesianOffsetUnits=mm  TranslationStandardAxis=+Z  TranslationStandardOffset=0  TranslationStandardOffsetUnits=m  TranslationROffset=0  TranslationROffsetUnits=m  TranslationThetaOffset=0  TranslationThetaOffsetUnits=deg  TranslationZOffset=0  TranslationZOffsetUnits=m
  Transform2 : sm_lib/Frames and Transforms/Rigid Transform  RotationMethod=ArbitraryAxis  FollAlignAxisA=+X  BaseAlignAxisA=+Y  FollAlignAxisB=+Y  BaseAlignAxisB=+Z  RotationStandardAxis=+Z  RotationAngle=smiData.RigidTransform(48).angle  RotationAngleUnits=rad  RotationArbitraryAxis=smiData.RigidTransform(48).axis  RotationSequenceAxes=FollowerAxes  RotationSequence=XYX  RotationSequenceAngles=[0 0 0]  RotationSequenceAnglesUnits=deg  RotationMatrix=[1 0 0;0 1 0;0 0 1]  Quaternion=[1 0 0 0]  TranslationMethod=Cartesian  TranslationCartesianOffset=smiData.RigidTransform(48).translation  TranslationCartesianOffsetUnits=mm  TranslationStandardAxis=+Z  TranslationStandardOffset=0  TranslationStandardOffsetUnits=m  TranslationROffset=0  TranslationROffsetUnits=m  TranslationThetaOffset=0  TranslationThetaOffsetUnits=deg  TranslationZOffset=0  TranslationZOffsetUnits=m
  F2 : PMIOPort  Side=Left
  F1 : PMIOPort  Port=2  Side=Right
  F : PMIOPort  Port=3  Side=Right
  connections:
  Solid/RConn1 -- ReferenceFrame/RConn1 -- Transform/LConn1 -- Transform1/LConn1 -- Transform2/LConn1
  Transform/RConn1 -- F/RConn1
  Transform1/RConn1 -- F1/RConn1
  Transform2/RConn1 -- F2/RConn1

== system mano_buena_pinza_paper/Abduccion_4/Esl41_RIGID ==
  ReferenceFrame : sm_lib/Frames and Transforms/Reference Frame
  Solid : sm_lib/Body Elements/File Solid  ExtGeomFileName=Esl4_ipt_c84328c3.STEP  UnitType=FromFile  ExtGeomFileUnits=m  StepReaderType=HEX  ExportConvexHullGeometry=off  InertiaType=Custom  BasedOnType=DensityFromFile  Density=1000  DensityUnits=kg/m^3  Mass=smiData.Solid(30).mass  MassUnits=kg  CenterOfMass=smiData.Solid(30).CoM  CenterOfMassUnits=mm  MomentsOfInertia=smiData.Solid(30).MoI  MomentsOfInertiaUnits=kg*mm^2  ProductsOfInertia=smiData.Solid(30).PoI  ProductsOfInertiaUnits=kg*mm^2  GraphicType=FromGeometry  MarkerShape=Sphere  MarkerSize=10  GraphicVisPropType=SimpleVisualProperties  GraphicDiffuseColor=smiData.Solid(30).color  GraphicOpacity=smiData.Solid(30).opacity  GraphicSpecularColor=[0.5 0.5 0.5 1.0]  GraphicAmbientColor=[0.15 0.15 0.15 1.0]  GraphicEmissiveColor=[0.0 0.0 0.0 1.0]  GraphicShininess=75  DoExposeReferenceFrame=on  SerializedFrames=<Frames/>
  Transform : sm_lib/Frames and Transforms/Rigid Transform  RotationMethod=ArbitraryAxis  FollAlignAxisA=+X  BaseAlignAxisA=+Y  FollAlignAxisB=+Y  BaseAlignAxisB=+Z  RotationStandardAxis=+Z  RotationAngle=smiData.RigidTransform(46).angle  RotationAngleUnits=rad  RotationArbitraryAxis=smiData.RigidTransform(46).axis  RotationSequenceAxes=FollowerAxes  RotationSequence=XYX  RotationSequenceAngles=[0 0 0]  RotationSequenceAnglesUnits=deg  RotationMatrix=[1 0 0;0 1 0;0 0 1]  Quaternion=[1 0 0 0]  TranslationMethod=Cartesian  TranslationCartesianOffset=smiData.RigidTransform(46).translation  TranslationCartesianOffsetUnits=mm  TranslationStandardAxis=+Z  TranslationStandardOffset=0  TranslationStandardOffsetUnits=m  TranslationROffset=0  TranslationROffsetUnits=m  TranslationThetaOffset=0  TranslationThetaOffsetUnits=deg  TranslationZOffset=0  TranslationZOffsetUnits=m
  Transform1 : sm_lib/Frames and Transforms/Rigid Transform  RotationMethod=ArbitraryAxis  FollAlignAxisA=+X  BaseAlignAxisA=+Y  FollAlignAxisB=+Y  BaseAlignAxisB=+Z  RotationStandardAxis=+Z  RotationAngle=smiData.RigidTransform(50).angle  RotationAngleUnits=rad  RotationArbitraryAxis=smiData.RigidTransform(50).axis  RotationSequenceAxes=FollowerAxes  RotationSequence=XYX  RotationSequenceAngles=[0 0 0]  RotationSequenceAnglesUnits=deg  RotationMatrix=[1 0 0;0 1 0;0 0 1]  Quaternion=[1 0 0 0]  TranslationMethod=Cartesian  TranslationCartesianOffset=smiData.RigidTransform(50).translation  TranslationCartesianOffsetUnits=mm  TranslationStandardAxis=+Z  TranslationStandardOffset=0  TranslationStandardOffsetUnits=m  TranslationROffset=0  TranslationROffsetUnits=m  TranslationThetaOffset=0  TranslationThetaOffsetUnits=deg  TranslationZOffset=0  TranslationZOffsetUnits=m
  F1 : PMIOPort  Side=Left
  F : PMIOPort  Port=2  Side=Left
  connections:
  Solid/RConn1 -- ReferenceFrame/RConn1 -- Transform/LConn1 -- Transform1/LConn1
  Transform/RConn1 -- F/RConn1
  Transform1/RConn1 -- F1/RConn1

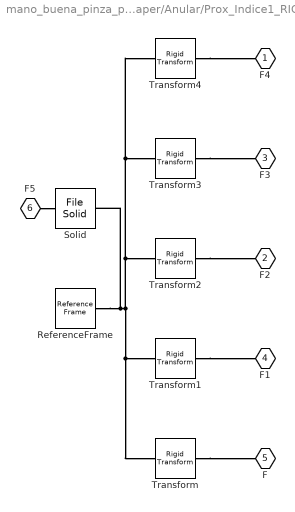
== system mano_buena_pinza_paper/Anular/Prox_Indice1_RIGID ==
  ReferenceFrame : sm_lib/Frames and Transforms/Reference Frame
  Solid : sm_lib/Body Elements/File Solid  ExtGeomFileName=Prox_Indice_ipt_552c8f7.STEP  UnitType=FromFile  ExtGeomFileUnits=m  StepReaderType=HEX  ExportConvexHullGeometry=on  InertiaType=Custom  BasedOnType=DensityFromFile  Density=1000  DensityUnits=kg/m^3  Mass=smiData.Solid(15).mass  MassUnits=kg  CenterOfMass=smiData.Solid(15).CoM  CenterOfMassUnits=mm  MomentsOfInertia=smiData.Solid(15).MoI  MomentsOfInertiaUnits=kg*mm^2  ProductsOfInertia=smiData.Solid(15).PoI  ProductsOfInertiaUnits=kg*mm^2  GraphicType=FromGeometry  MarkerShape=Sphere  MarkerSize=10  GraphicVisPropType=SimpleVisualProperties  GraphicDiffuseColor=smiData.Solid(15).color  GraphicOpacity=smiData.Solid(15).opacity  GraphicSpecularColor=[0.5 0.5 0.5 1.0]  GraphicAmbientColor=[0.15 0.15 0.15 1.0]  GraphicEmissiveColor=[0.0 0.0 0.0 1.0]  GraphicShininess=75  DoExposeReferenceFrame=on  SerializedFrames=<Frames/>
  Transform : sm_lib/Frames and Transforms/Rigid Transform  RotationMethod=ArbitraryAxis  FollAlignAxisA=+X  BaseAlignAxisA=+Y  FollAlignAxisB=+Y  BaseAlignAxisB=+Z  RotationStandardAxis=+Z  RotationAngle=smiData.RigidTransform(9).angle  RotationAngleUnits=rad  RotationArbitraryAxis=smiData.RigidTransform(9).axis  RotationSequenceAxes=FollowerAxes  RotationSequence=XYX  RotationSequenceAngles=[0 0 0]  RotationSequenceAnglesUnits=deg  RotationMatrix=[1 0 0;0 1 0;0 0 1]  Quaternion=[1 0 0 0]  TranslationMethod=Cartesian  TranslationCartesianOffset=smiData.RigidTransform(9).translation  TranslationCartesianOffsetUnits=mm  TranslationStandardAxis=+Z  TranslationStandardOffset=0  TranslationStandardOffsetUnits=m  TranslationROffset=0  TranslationROffsetUnits=m  TranslationThetaOffset=0  TranslationThetaOffsetUnits=deg  TranslationZOffset=0  TranslationZOffsetUnits=m
  Transform1 : sm_lib/Frames and Transforms/Rigid Transform  RotationMethod=ArbitraryAxis  FollAlignAxisA=+X  BaseAlignAxisA=+Y  FollAlignAxisB=+Y  BaseAlignAxisB=+Z  RotationStandardAxis=+Z  RotationAngle=smiData.RigidTransform(13).angle  RotationAngleUnits=rad  RotationArbitraryAxis=smiData.RigidTransform(13).axis  RotationSequenceAxes=FollowerAxes  RotationSequence=XYX  RotationSequenceAngles=[0 0 0]  RotationSequenceAnglesUnits=deg  RotationMatrix=[1 0 0;0 1 0;0 0 1]  Quaternion=[1 0 0 0]  TranslationMethod=Cartesian  TranslationCartesianOffset=smiData.RigidTransform(13).translation  TranslationCartesianOffsetUnits=mm  TranslationStandardAxis=+Z  TranslationStandardOffset=0  TranslationStandardOffsetUnits=m  TranslationROffset=0  TranslationROffsetUnits=m  TranslationThetaOffset=0  TranslationThetaOffsetUnits=deg  TranslationZOffset=0  TranslationZOffsetUnits=m
  Transform2 : sm_lib/Frames and Transforms/Rigid Transform  RotationMethod=ArbitraryAxis  FollAlignAxisA=+X  BaseAlignAxisA=+Y  FollAlignAxisB=+Y  BaseAlignAxisB=+Z  RotationStandardAxis=+Z  RotationAngle=smiData.RigidTransform(58).angle  RotationAngleUnits=rad  RotationArbitraryAxis=smiData.RigidTransform(58).axis  RotationSequenceAxes=FollowerAxes  RotationSequence=XYX  RotationSequenceAngles=[0 0 0]  RotationSequenceAnglesUnits=deg  RotationMatrix=[1 0 0;0 1 0;0 0 1]  Quaternion=[1 0 0 0]  TranslationMethod=Cartesian  TranslationCartesianOffset=smiData.RigidTransform(58).translation  TranslationCartesianOffsetUnits=mm  TranslationStandardAxis=+Z  TranslationStandardOffset=0  TranslationStandardOffsetUnits=m  TranslationROffset=0  TranslationROffsetUnits=m  TranslationThetaOffset=0  TranslationThetaOffsetUnits=deg  TranslationZOffset=0  TranslationZOffsetUnits=m
  Transform3 : sm_lib/Frames and Transforms/Rigid Transform  RotationMethod=ArbitraryAxis  FollAlignAxisA=+X  BaseAlignAxisA=+Y  FollAlignAxisB=+Y  BaseAlignAxisB=+Z  RotationStandardAxis=+Z  RotationAngle=smiData.RigidTransform(73).angle  RotationAngleUnits=rad  RotationArbitraryAxis=smiData.RigidTransform(73).axis  RotationSequenceAxes=FollowerAxes  RotationSequence=XYX  RotationSequenceAngles=[0 0 0]  RotationSequenceAnglesUnits=deg  RotationMatrix=[1 0 0;0 1 0;0 0 1]  Quaternion=[1 0 0 0]  TranslationMethod=Cartesian  TranslationCartesianOffset=smiData.RigidTransform(73).translation  TranslationCartesianOffsetUnits=mm  TranslationStandardAxis=+Z  TranslationStandardOffset=0  TranslationStandardOffsetUnits=m  TranslationROffset=0  TranslationROffsetUnits=m  TranslationThetaOffset=0  TranslationThetaOffsetUnits=deg  TranslationZOffset=0  TranslationZOffsetUnits=m
  Transform4 : sm_lib/Frames and Transforms/Rigid Transform  RotationMethod=ArbitraryAxis  FollAlignAxisA=+X  BaseAlignAxisA=+Y  FollAlignAxisB=+Y  BaseAlignAxisB=+Z  RotationStandardAxis=+Z  RotationAngle=smiData.RigidTransform(102).angle  RotationAngleUnits=rad  RotationArbitraryAxis=smiData.RigidTransform(102).axis  RotationSequenceAxes=FollowerAxes  RotationSequence=XYX  RotationSequenceAngles=[0 0 0]  RotationSequenceAnglesUnits=deg  RotationMatrix=[1 0 0;0 1 0;0 0 1]  Quaternion=[1 0 0 0]  TranslationMethod=Cartesian  TranslationCartesianOffset=smiData.RigidTransform(102).translation  TranslationCartesianOffsetUnits=mm  TranslationStandardAxis=+Z  TranslationStandardOffset=0  TranslationStandardOffsetUnits=m  TranslationROffset=0  TranslationROffsetUnits=m  TranslationThetaOffset=0  TranslationThetaOffsetUnits=deg  TranslationZOffset=0  TranslationZOffsetUnits=m
  F4 : PMIOPort  Side=Left
  F2 : PMIOPort  Port=2  Side=Left
  F3 : PMIOPort  Port=3  Side=Right
  F1 : PMIOPort  Port=4  Side=Right
  F : PMIOPort  Port=5  Side=Right
  F5 : PMIOPort  Port=6  Side=Right
  connections:
  Solid/RConn1 -- ReferenceFrame/RConn1 -- Transform/LConn1 -- Transform1/LConn1 -- Transform3/LConn1 -- Transform4/LConn1 -- Transform2/LConn1
  Transform/RConn1 -- F/RConn1
  Transform1/RConn1 -- F1/RConn1
  Transform2/RConn1 -- F2/RConn1
  Transform3/RConn1 -- F3/RConn1
  Transform4/RConn1 -- F4/RConn1
  F5/RConn1 -- Solid/LConn1

== system mano_buena_pinza_paper/Anular/Tapa_prox_medio1_RIGID ==
  ReferenceFrame : sm_lib/Frames and Transforms/Reference Frame
  Solid : sm_lib/Body Elements/File Solid  ExtGeomFileName=Tapa_prox_medio_ipt_ad682b4a.STEP  UnitType=FromFile  ExtGeomFileUnits=m  StepReaderType=HEX  ExportConvexHullGeometry=off  InertiaType=Custom  BasedOnType=DensityFromFile  Density=1000  DensityUnits=kg/m^3  Mass=smiData.Solid(16).mass  MassUnits=kg  CenterOfMass=smiData.Solid(16).CoM  CenterOfMassUnits=mm  MomentsOfInertia=smiData.Solid(16).MoI  MomentsOfInertiaUnits=kg*mm^2  ProductsOfInertia=smiData.Solid(16).PoI  ProductsOfInertiaUnits=kg*mm^2  GraphicType=FromGeometry  MarkerShape=Sphere  MarkerSize=10  GraphicVisPropType=SimpleVisualProperties  GraphicDiffuseColor=smiData.Solid(16).color  GraphicOpacity=smiData.Solid(16).opacity  GraphicSpecularColor=[0.5 0.5 0.5 1.0]  GraphicAmbientColor=[0.15 0.15 0.15 1.0]  GraphicEmissiveColor=[0.0 0.0 0.0 1.0]  GraphicShininess=75  DoExposeReferenceFrame=on  SerializedFrames=<Frames/>
  Transform : sm_lib/Frames and Transforms/Rigid Transform  RotationMethod=ArbitraryAxis  FollAlignAxisA=+X  BaseAlignAxisA=+Y  FollAlignAxisB=+Y  BaseAlignAxisB=+Z  RotationStandardAxis=+Z  RotationAngle=smiData.RigidTransform(101).angle  RotationAngleUnits=rad  RotationArbitraryAxis=smiData.RigidTransform(101).axis  RotationSequenceAxes=FollowerAxes  RotationSequence=XYX  RotationSequenceAngles=[0 0 0]  RotationSequenceAnglesUnits=deg  RotationMatrix=[1 0 0;0 1 0;0 0 1]  Quaternion=[1 0 0 0]  TranslationMethod=Cartesian  TranslationCartesianOffset=smiData.RigidTransform(101).translation  TranslationCartesianOffsetUnits=mm  TranslationStandardAxis=+Z  TranslationStandardOffset=0  TranslationStandardOffsetUnits=m  TranslationROffset=0  TranslationROffsetUnits=m  TranslationThetaOffset=0  TranslationThetaOffsetUnits=deg  TranslationZOffset=0  TranslationZOffsetUnits=m
  F : PMIOPort  Side=Left
  connections:
  Solid/RConn1 -- ReferenceFrame/RConn1 -- Transform/LConn1
  Transform/RConn1 -- F/RConn1
